simulink model "Bossi_Emanuele_EE460S3D_R99"  (R2025a)
settings: Solver=FixedStepDiscrete  StartTime=0.0  StopTime=120  FixedStep=dt0  RelTol=1e-3  EnableMultiTasking=on
PostLoadFcn:
  | %Set the size for the model
  | set_param(gcs,'Location',[10 10 1270 970])
  | %Set the zoom factor for the model
  | set_param(gcs,'ZoomFactor','100')
InitFcn:
  | tic
  | Bossi_Emanuele_EE460_Final
  | INIT_S3D_01
StartFcn:
  | tend0=toc;
  | tic;
StopFcn:
  | tend=toc;
  | disp(['Simulation time = ' num2str(tout(end)) ' sec'])
  | disp(['Real time = ' num2str(tend) ' sec'])
  | title('DONE')
  | SCORE=round((max(0,120-tout(end)-tend0))*4+10*(40-FuelBurned)+sum(100*double(PDONE)-100*double(PDONE<.5)));
  | PlotS3D(PlotInput);
  | text(15,22,['S: ' num2str(SCORE)]);
  | % Reset color scheme back to normal defaults
  | figure()
  | blkwhitebg('w');
  | close
values from neighbouring files (symbols this model uses):
  A_obs = [ 0  1  0  0  0  0 ... (first row only)    [Bossi_Emanuele_EE460_Final.m]
  B_obs = [ 0     0     0 ... (first row only)    [Bossi_Emanuele_EE460_Final.m]
  C_obs = [ 1 0 0 0 0 0 ... (first row only)    [Bossi_Emanuele_EE460_Final.m]
  d2r = pi/180    (= 0.0174532925199)    [INIT_S3D_01.m]
  D_obs = [ 0     0     0 ... (first row only)    [Bossi_Emanuele_EE460_Final.m]
  dt = 0.01    [INIT_S3D_01.m]
  dt0 = 0.001    [INIT_S3D_01.m]
  fr = 100    [INIT_S3D_01.m]
  G = [1,  1, -1, -1,  0,  0,  0,  0 ... (first row only)    [Bossi_Emanuele_EE460_Final.m]
  G_obs = eye(6)    [Bossi_Emanuele_EE460_Final.m]
  HM_S = 250    [INIT_S3D_01.m]
  HM_U = 500    [INIT_S3D_01.m]
  J = Jbase+JC0+JF+M*(Xcg^2+Ycg^2)    [INIT_S3D_01.m]
  Jbase = JC1+4*Ja+2*Ma*da^2+2*Ma*db^2    [INIT_S3D_01.m]
  JC0 = MC0/2    (= 10.2101761242)    [INIT_S3D_01.m]
  Kdtheta = 2 * zeta_th * wn_th * J_eff    [Bossi_Emanuele_EE460_Final.m]
  Kdtheta_fail = 2 * zeta_th_fail * wn_th_fail * J_eff    [Bossi_Emanuele_EE460_Final.m]
  Kdx = 2 * zeta_xy * wn_xy * M_eff    [Bossi_Emanuele_EE460_Final.m]
  Kdx_fail = 2 * zeta_xy_fail * wn_xy_fail * M_eff    [Bossi_Emanuele_EE460_Final.m]
  Kdy = 2 * zeta_xy * wn_xy * M_eff    [Bossi_Emanuele_EE460_Final.m]
  Kdy_fail = 2 * zeta_xy_fail * wn_xy_fail * M_eff    [Bossi_Emanuele_EE460_Final.m]
  Kptheta = J_eff * wn_th^2    [Bossi_Emanuele_EE460_Final.m]
  Kptheta_fail = J_eff * wn_th_fail^2    [Bossi_Emanuele_EE460_Final.m]
  Kpx = M_eff * wn_xy^2    [Bossi_Emanuele_EE460_Final.m]
  Kpx_fail = M_eff * wn_xy_fail^2    [Bossi_Emanuele_EE460_Final.m]
  Kpy = M_eff * wn_xy^2    [Bossi_Emanuele_EE460_Final.m]
  Kpy_fail = M_eff * wn_xy_fail^2    [Bossi_Emanuele_EE460_Final.m]
  L13 = sqrt(10)    [INIT_S3D_01.m]
  L24 = sqrt(6.25)    [INIT_S3D_01.m]
  LVL = LVL12    [INIT_S3D_01.m]
  M = MC+M1+M2+M3+M4+4*Ma    [INIT_S3D_01.m]
  M1 = LVL.M1    [INIT_S3D_01.m]
  M2 = LVL.M2    [INIT_S3D_01.m]
  M3 = LVL.M3    [INIT_S3D_01.m]
  M4 = LVL.M4    [INIT_S3D_01.m]
  max_qddot = [max_qddot_x; max_qddot_y; max_qddot_theta]    [Bossi_Emanuele_EE460_Final.m]
  mdti = (1/300)    (= 0.00333333333333)    [INIT_S3D_01.m]
  P = [1  1 -1 -1  0  0  0  0 ... (first row only)    [Bossi_Emanuele_EE460_Final.m]
  Pdata = [LVL.P1 LVL.P2 LVL.P3 LVL.P4]    [INIT_S3D_01.m]    (also in PlotS3D.m = R*[xt1;yt1+[0 3*tt*TV(idx-13)*TSIG(idx-13) 0]])
  PTvec = [Pdata(:,1);Pdata(:,2);Pdata(:,3);Pdata(:,4) ... (first row only)    [INIT_S3D_01.m]
  Q_obs = eye(6)    [Bossi_Emanuele_EE460_Final.m]
  r2d = 180/pi    (= 57.2957795131)    [INIT_S3D_01.m]
  r_bang = 0.5    [Bossi_Emanuele_EE460_Final.m]
  Sconfig = 1    [Bossi_Emanuele_EE460_Final.m]
  SLIM = [-100 100 ... (first row only)    [INIT_S3D_01.m]
  SQ = [.005 .01 .004 .005 .01 .004 .02 .01 .4]'    [INIT_S3D_01.m]
  SSF = 1./SQ    [INIT_S3D_01.m]
  tau = 0.5    [Bossi_Emanuele_EE460_Final.m]
  TOLdata = [LVL.P1tol LVL.P2tol LVL.P3tol LVL.P4tol]    [INIT_S3D_01.m]
  ULIM = [[Umin Umax];0 0;0 0]    [INIT_S3D_01.m]
undefined symbols (not defined in the file or in its folder): den_lp, den_lp2, DiscIntNeverNeededParam, dt1_bang_3, dt2_bang_3, dtc_bang_3, num_lp, num_lp2, q0_1
libraries: simulink x87, matrix_library x4, sl3dlib x1, aerolibutil x1, aerolibanimutils x1
(part 8 of 8)

== system Bossi_Emanuele_EE460S3D_R99/S3D_Plant/ThrusterValues/HealthMonitoring/DetectFailures/Subsystem9 ==
  UCMD : Inport
  U : Inport  Port=2
  Abs : Abs  SaturateOnIntegerOverflow=off
  Compare To Constant : simulink/Logic and Bit Operations/Compare To Constant  relop=>=  const=HM_U  OutDataTypeStr=boolean
  Constant : Constant  Value=0
  Constant1 : Constant
  Logical Operator : Logic  Operator=OR  AllPortsSameDT=off  OutDataTypeStr=boolean
  Signal Specification : SignalSpecification  Dimensions=[1]
  Signal Specification1 : SignalSpecification  Dimensions=[1]
  Sum : Sum  Inputs=|+-
  Sum1 : Sum  Inputs=++|
  Switch : Switch  Criteria=u2 > Threshold  Threshold=.4  SaturateOnIntegerOverflow=off  InputSameDT=off
  Unit Delay1 : UnitDelay  SampleTime=dt0  HasFrameUpgradeWarning=on
  Unit Delay2 : UnitDelay  SampleTime=dt0  HasFrameUpgradeWarning=on
  Out1 : Outport
  wires:
  Abs/1 -> Switch/2
  Signal Specification1/1 -> Sum/2
  Signal Specification/1 -> Sum/1
  Constant/1 -> Switch/3
  Sum1/1 -> Switch/1
  Unit Delay1/1 -> Sum1/1
  Constant1/1 -> Sum1/2
  U/1 -> Signal Specification1/1
  Logical Operator/1 -> Unit Delay2/1, Out1/1
  Compare To Constant/1 -> Logical Operator/1
  Switch/1 -> Unit Delay1/1, Compare To Constant/1
  UCMD/1 -> Signal Specification/1
  Unit Delay2/1 -> Logical Operator/2
  Sum/1 -> Abs/1

== system Bossi_Emanuele_EE460S3D_R99/ControlLaw/Command/AutoMode/BangBang_cmd/Precomputations/ComputeBCBTimes ==
  CurrentPosition1 : Inport
  In2 : Inport  Port=2
  FinalPosition1 : Inport  Port=3
  CurrentVelocity : Inport  Port=4
  Bus Creator : BusCreator  Inputs=3
  Bus Creator1 : BusCreator  Inputs=6
  Bus Selector : BusSelector  OutputSignals=FinalPosition,TriggeredPosition,a
  Constant : Constant  Value=r_bang  SampleTime=dt
  Constant1 : Constant
  Constant3 : Constant  Value=r_bang  SampleTime=dt
  DeltaQ : Subsystem
  Demux : Demux  Outputs=3
  Demux1 : Demux  Outputs=3
  Demux2 : Demux  Outputs=3
  Gain : Gain  Gain=2
  Max : MinMax  Function=max  Inputs=3
  Product : Product
  Product1 : Product
  RecomputeAccelerations : Subsystem
  Subsystem : Subsystem
  Sum1 : Sum  Inputs=|++
  Sum2 : Sum  Inputs=++|
  Sum3 : Sum  Inputs=++|
  Out4 : Outport
  Out1 : Outport  Port=2
  Out3 : Outport  Port=3
  Acc : Outport  Port=4
  wires:
  CurrentPosition1/1 -> Bus Creator/1
  In2/1 -> Bus Creator/2  "a"
  FinalPosition1/1 -> Bus Creator/3
  Bus Creator/1 -> Bus Selector/1
  Bus Selector/1 -> Demux1/1  "<FinalPosition>"
  Bus Selector/2 -> Demux2/1  "<TriggeredPosition>"
  DeltaQ/1(DeltaQ) -> RecomputeAccelerations/1(DeltaQ), Subsystem/2(DeltaQ)  "DeltaQ"
  Constant/1 -> Sum1/1
  Constant1/1 -> Sum1/2
  Bus Selector/3 -> Subsystem/3(Acc), Gain/1  "<a>"
  Sum1/1 -> Product/2
  Product/1 -> Subsystem/4(Den)  "rPlusOne"
  Subsystem/1(Out1) -> Demux/1
  Demux/2 -> Max/2
  Demux/1 -> Max/1
  Demux/3 -> Max/3
  Max/1 -> Product1/1, Sum2/2, RecomputeAccelerations/3(dt1), Sum3/1, Out1/1  "dt"
  Constant3/1 -> Product1/2
  Sum2/1 -> Out4/1  "TF"
  Product1/1 -> Sum3/2  "dtc"
  Sum3/1 -> Out3/1, Sum2/1  "DtPlusDtc"
  RecomputeAccelerations/1(Acc) -> Acc/1
  Demux1/1 -> Bus Creator1/1
  Demux1/2 -> Bus Creator1/2
  Demux1/3 -> Bus Creator1/3
  Demux2/1 -> Bus Creator1/4
  Demux2/2 -> Bus Creator1/5
  Demux2/3 -> Bus Creator1/6
  Bus Creator1/1 -> DeltaQ/1(In1)  "positions"
  Gain/1 -> Product/1
  CurrentVelocity/1 -> RecomputeAccelerations/2(v0), Subsystem/1(CurrentVelocity)

== system Bossi_Emanuele_EE460S3D_R99/ControlLaw/Command/AutoMode/BangBang_cmd/Precomputations/VariableTimer ==
  In1 : Inport
  Constant : Constant  Value=dt
  DetectTFchange : Subsystem
  Logical Operator : Logic  Operator=OR  AllPortsSameDT=off  OutDataTypeStr=boolean
  Relational Operator : RelationalOperator  Operator=<=  OutDataTypeStr=boolean  RndMeth=Simplest  InputSameDT=off
  Sum : Sum  Inputs=|++
  Switch : Switch  Criteria=u2 > Threshold  SaturateOnIntegerOverflow=off  InputSameDT=off
  Unit Delay1 : UnitDelay  SampleTime=dt  HasFrameUpgradeWarning=on
  Unit Delay2 : UnitDelay  InitialCondition=-dt  SampleTime=dt  HasFrameUpgradeWarning=on
  Time_sec : Outport
  wires:
  Unit Delay2/1 -> Sum/2
  Sum/1 -> Relational Operator/2, Switch/3
  Constant/1 -> Sum/1
  Logical Operator/1 -> Switch/2
  Switch/1 -> Time_sec/1, Unit Delay1/1, Unit Delay2/1  "Time_sec"
  DetectTFchange/1(Out1) -> Switch/1
  Unit Delay1/1 -> DetectTFchange/1(In1)  "TimeZ_sec"
  DetectTFchange/2(Out2) -> Logical Operator/1
  In1/1 -> DetectTFchange/2(In3), Relational Operator/1
  Relational Operator/1 -> Logical Operator/2  "Reset1"

== system Bossi_Emanuele_EE460S3D_R99/ControlLaw/Command/AutoMode/BangBang_cmd/ThetaTargetCorrector/AngleWrapper ==
  In1 : Inport
  Atan2 : Trigonometry  Operator=atan2
  Cos : Trigonometry  Operator=cos
  Gain : Gain  Gain=180/pi
  Gain6 : Gain  Gain=pi/180
  Sin : Trigonometry
  Out1 : Outport
  wires:
  Gain6/1 -> Cos/1, Sin/1
  In1/1 -> Gain6/1
  Atan2/1 -> Gain/1
  Gain/1 -> Out1/1  "WrappedAngle_deg"
  Sin/1 -> Atan2/1
  Cos/1 -> Atan2/2

== system Bossi_Emanuele_EE460S3D_R99/ControlLaw/Command/InitialPoint/BangBang_cmd/Precomputations/ComputeBCBTimes ==
  CurrentPosition1 : Inport
  In2 : Inport  Port=2
  Abs : Abs  SaturateOnIntegerOverflow=off
  Bus Creator : BusCreator  Inputs=3
  Bus Creator1 : BusCreator  Inputs=6
  Bus Selector : BusSelector  OutputSignals=FinalPosition,TriggeredPosition,a
  Constant : Constant  Value=r_bang  SampleTime=dt
  Constant1 : Constant
  Constant2 : Constant  Value=0.5  SampleTime=dt
  Constant3 : Constant  Value=r_bang  SampleTime=dt
  Constant4 : Constant  Value=[0; 0; 0]  SampleTime=dt
  DeltaQ : Subsystem
  Demux : Demux  Outputs=3
  Demux1 : Demux  Outputs=3
  Demux2 : Demux  Outputs=3
  Divide : Product  Inputs=*/
  Math Function : Math  Operator=pow
  Max : MinMax  Function=max  Inputs=3
  Product : Product
  Product1 : Product
  RecomputeAccelerations : Subsystem
  Sum1 : Sum  Inputs=|++
  Sum2 : Sum  Inputs=++|
  Sum3 : Sum  Inputs=++|
  Out4 : Outport
  Out1 : Outport  Port=2
  Out3 : Outport  Port=3
  Acc : Outport  Port=4
  wires:
  CurrentPosition1/1 -> Bus Creator/1
  In2/1 -> Bus Creator/2  "a"
  Bus Creator/1 -> Bus Selector/1
  Bus Selector/1 -> Demux1/1  "<FinalPosition>"
  Bus Selector/2 -> Demux2/1  "<TriggeredPosition>"
  DeltaQ/1(Out1) -> RecomputeAccelerations/1(In1), Divide/1  "DeltaQ"
  Constant/1 -> Sum1/1
  Constant1/1 -> Sum1/2
  Bus Selector/3 -> Product/1  "<a>"
  Sum1/1 -> Product/2
  Product/1 -> Divide/2  "rPlusOne"
  Constant2/1 -> Math Function/2
  Divide/1 -> Abs/1
  Math Function/1 -> Demux/1
  Demux/2 -> Max/2
  Demux/1 -> Max/1
  Demux/3 -> Max/3
  Max/1 -> Product1/1, Sum2/2, RecomputeAccelerations/2(In3), Sum3/1, Out1/1  "dt"
  Constant3/1 -> Product1/2
  Sum2/1 -> Out4/1  "TF"
  Product1/1 -> Sum3/2  "dtc"
  Sum3/1 -> Out3/1, Sum2/1  "DtPlusDtc"
  RecomputeAccelerations/1(Acc) -> Acc/1
  Demux1/1 -> Bus Creator1/1
  Demux1/2 -> Bus Creator1/2
  Demux1/3 -> Bus Creator1/3
  Demux2/1 -> Bus Creator1/4
  Demux2/2 -> Bus Creator1/5
  Demux2/3 -> Bus Creator1/6
  Bus Creator1/1 -> DeltaQ/1(In1)  "positions"
  Abs/1 -> Math Function/1
  Constant4/1 -> Bus Creator/3  "FinalPosition"

== system Bossi_Emanuele_EE460S3D_R99/ControlLaw/Command/InitialPoint/BangBang_cmd/Precomputations/VariableTimer ==
  In1 : Inport
  Constant : Constant  Value=dt
  DetectTFchange : Subsystem
  Logical Operator : Logic  Operator=OR  AllPortsSameDT=off  OutDataTypeStr=boolean
  Relational Operator : RelationalOperator  Operator=<=  OutDataTypeStr=boolean  RndMeth=Simplest  InputSameDT=off
  Sum : Sum  Inputs=|++
  Switch : Switch  Criteria=u2 > Threshold  SaturateOnIntegerOverflow=off  InputSameDT=off
  Unit Delay1 : UnitDelay  SampleTime=dt  HasFrameUpgradeWarning=on
  Unit Delay2 : UnitDelay  InitialCondition=-dt  SampleTime=dt  HasFrameUpgradeWarning=on
  Time_sec : Outport
  wires:
  Unit Delay2/1 -> Sum/2
  Sum/1 -> Relational Operator/2, Switch/3
  Constant/1 -> Sum/1
  Logical Operator/1 -> Switch/2
  Switch/1 -> Time_sec/1, Unit Delay1/1, Unit Delay2/1  "Time_sec"
  DetectTFchange/1(Out1) -> Switch/1
  Unit Delay1/1 -> DetectTFchange/1(In1)  "TimeZ_sec"
  DetectTFchange/2(Out2) -> Logical Operator/1
  In1/1 -> DetectTFchange/2(In3), Relational Operator/1
  Relational Operator/1 -> Logical Operator/2  "Reset1"

== system Bossi_Emanuele_EE460S3D_R99/ControlLaw/Command/InitialPoint/BangBang_cmd/ThetaTargetCorrector/AngleWrapper ==
  In1 : Inport
  Atan2 : Trigonometry  Operator=atan2
  Cos : Trigonometry  Operator=cos
  Gain : Gain  Gain=180/pi
  Gain6 : Gain  Gain=pi/180
  Sin : Trigonometry
  Out1 : Outport
  wires:
  Gain6/1 -> Cos/1, Sin/1
  In1/1 -> Gain6/1
  Atan2/1 -> Gain/1
  Gain/1 -> Out1/1  "WrappedAngle_deg"
  Sin/1 -> Atan2/1
  Cos/1 -> Atan2/2

== system Bossi_Emanuele_EE460S3D_R99/ControlLaw/Command/AutoMode/BangBang_cmd/Precomputations/ComputeBCBTimes/DeltaQ ==
  In1 : Inport
  Bus Selector1 : BusSelector  OutputSignals=signal1,signal4,signal2,signal5,signal3,signal6
  Display : Display
  Sum : Sum  Inputs=|+-
  Sum4 : Sum  Inputs=|+-
  ThetaTargetCorrector : Subsystem
  Vector Concatenate : Concatenate  NumInputs=3
  DeltaQ : Outport
  wires:
  Bus Selector1/4 -> Sum4/2  "<signal5>"
  Bus Selector1/3 -> Sum4/1  "<signal2>"
  Sum4/1 -> Vector Concatenate/2  "DeltaY"
  Bus Selector1/1 -> Sum/1  "<signal1>"
  Bus Selector1/2 -> Sum/2  "<signal4>"
  Bus Selector1/5 -> ThetaTargetCorrector/1(In2)  "<signal3>"
  ThetaTargetCorrector/1(Out1) -> Vector Concatenate/3  "qc"
  Bus Selector1/6 -> ThetaTargetCorrector/2(In1)  "<signal6>"
  Sum/1 -> Display/1, Vector Concatenate/1  "DeltaX"
  In1/1 -> Bus Selector1/1
  Vector Concatenate/1 -> DeltaQ/1  "DeltaQ"

== system Bossi_Emanuele_EE460S3D_R99/ControlLaw/Command/AutoMode/BangBang_cmd/Precomputations/ComputeBCBTimes/RecomputeAccelerations ==
  DeltaQ : Inport
  v0 : Inport  Port=2
  dt1 : Inport  Port=3
  Constant : Constant  Value=r_bang  SampleTime=dt
  Constant1 : Constant  Value=r_bang  SampleTime=dt
  Constant2 : Constant  Value=2
  Constant3 : Constant
  Constant4 : Constant  Value=2
  Divide : Product  Inputs=*/
  Pow : Math  Operator=pow  SignedPower=on  RndMeth=Zero
  Product : Product  Inputs=3
  Product1 : Product
  Sum : Sum  Inputs=|++
  Sum1 : Sum  Inputs=|+-
  Sum2 : Sum  Inputs=|++
  Acc : Outport
  wires:
  Divide/1 -> Acc/1  "a"
  Constant2/1 -> Sum/1
  Constant/1 -> Sum/2
  Sum/1 -> Product/2
  v0/1 -> Product/1
  dt1/1 -> Pow/1, Product/3
  DeltaQ/1 -> Sum1/1
  Sum1/1 -> Divide/1
  Product/1 -> Sum1/2
  Constant1/1 -> Sum2/2
  Constant3/1 -> Sum2/1
  Sum2/1 -> Product1/2
  Pow/1 -> Product1/1
  Constant4/1 -> Pow/2
  Product1/1 -> Divide/2

== system Bossi_Emanuele_EE460S3D_R99/ControlLaw/Command/AutoMode/BangBang_cmd/Precomputations/ComputeBCBTimes/Subsystem ==
  CurrentVelocity : Inport
  DeltaQ : Inport  Port=2
  Acc : Inport  Port=3
  Den : Inport  Port=4
  Abs : Abs  SaturateOnIntegerOverflow=off
  Bus Creator : BusCreator  Inputs=2
  Bus Selector : BusSelector  OutputSignals=NegVelZero,TwoPlusR,NegVelZero,TwoPlusR
  Constant : Constant  Value=r_bang  SampleTime=dt
  Constant1 : Constant  Value=2
  Constant2 : Constant  Value=2
  Constant3 : Constant  Value=2
  Constant4 : Constant  Value=r_bang  SampleTime=dt
  Constant5 : Constant
  Constant6 : Constant  Value=0.5
  Divide : Product  Inputs=*/
  Exp : Math  Operator=pow
  Exp1 : Math  Operator=pow
  Gain : Gain  Gain=-1
  Gain1 : Gain  Gain=4
  Pow : Math  Operator=pow  SignedPower=on  RndMeth=Zero
  Product : Product
  Product1 : Product
  Product2 : Product  Inputs=3
  Sum : Sum  Inputs=|++
  Sum1 : Sum  Inputs=|++
  Sum2 : Sum  Inputs=|++|
  Sum3 : Sum  Inputs=|++
  Out1 : Outport
  wires:
  CurrentVelocity/1 -> Gain/1
  Constant/1 -> Sum/1
  Constant1/1 -> Sum/2
  Gain/1 -> Bus Creator/1  "NegVelZero"
  Sum/1 -> Bus Creator/2  "TwoPlusR"
  Bus Creator/1 -> Bus Selector/1
  Bus Selector/1 -> Product/1  "<NegVelZero>"
  Bus Selector/2 -> Product/2  "<TwoPlusR>"
  Bus Selector/3 -> Exp/1  "<NegVelZero>"
  Constant2/1 -> Exp/2
  Bus Selector/4 -> Exp1/1  "<TwoPlusR>"
  Constant3/1 -> Exp1/2
  Exp/1 -> Product1/1
  Exp1/1 -> Product1/2
  Product1/1 -> Sum1/1
  Constant5/1 -> Sum2/2
  Constant4/1 -> Sum2/1
  Acc/1 -> Gain1/1
  Gain1/1 -> Product2/1
  Sum2/1 -> Product2/2  "TwoPlusR"
  DeltaQ/1 -> Product2/3
  Product2/1 -> Sum1/2
  Sum1/1 -> Abs/1
  Abs/1 -> Pow/1
  Constant6/1 -> Pow/2
  Pow/1 -> Sum3/2
  Product/1 -> Sum3/1
  Sum3/1 -> Divide/1
  Den/1 -> Divide/2
  Divide/1 -> Out1/1  "t1"

== system Bossi_Emanuele_EE460S3D_R99/ControlLaw/Command/AutoMode/BangBang_cmd/Precomputations/VariableTimer/DetectTFchange ==
  In1 : Inport
  In3 : Inport  Port=2
  Constant : Constant  Value=0
  Relational Operator1 : RelationalOperator  Operator=~=  OutDataTypeStr=boolean  RndMeth=Simplest  InputSameDT=off
  Switch3 : Switch  Criteria=u2 > Threshold  SaturateOnIntegerOverflow=off  InputSameDT=off
  Unit Delay : UnitDelay  InitialCondition=-dt  SampleTime=dt  HasFrameUpgradeWarning=on
  Out1 : Outport
  Out2 : Outport  Port=2
  wires:
  Switch3/1 -> Out1/1  "ResetValue"
  In3/1 -> Relational Operator1/1, Unit Delay/1
  Unit Delay/1 -> Relational Operator1/2
  Relational Operator1/1 -> Out2/1, Switch3/2  "Reset2"
  In1/1 -> Switch3/3
  Constant/1 -> Switch3/1

== system Bossi_Emanuele_EE460S3D_R99/ControlLaw/Command/InitialPoint/BangBang_cmd/Precomputations/ComputeBCBTimes/DeltaQ ==
  In1 : Inport
  Bus Selector1 : BusSelector  OutputSignals=signal1,signal4,signal2,signal5,signal3,signal6
  Display : Display
  Sum : Sum  Inputs=|+-
  Sum4 : Sum  Inputs=|+-
  ThetaTargetCorrector : Subsystem
  Vector Concatenate : Concatenate  NumInputs=3
  Out1 : Outport
  wires:
  Bus Selector1/4 -> Sum4/2  "<signal5>"
  Bus Selector1/3 -> Sum4/1  "<signal2>"
  Sum4/1 -> Vector Concatenate/2  "DeltaY"
  Bus Selector1/1 -> Sum/1  "<signal1>"
  Bus Selector1/2 -> Sum/2  "<signal4>"
  Bus Selector1/5 -> ThetaTargetCorrector/1(In2)  "<signal3>"
  ThetaTargetCorrector/1(Out1) -> Vector Concatenate/3  "qc"
  Bus Selector1/6 -> ThetaTargetCorrector/2(In1)  "<signal6>"
  Sum/1 -> Display/1, Vector Concatenate/1  "DeltaX"
  In1/1 -> Bus Selector1/1
  Vector Concatenate/1 -> Out1/1  "DeltaQ"

== system Bossi_Emanuele_EE460S3D_R99/ControlLaw/Command/InitialPoint/BangBang_cmd/Precomputations/ComputeBCBTimes/RecomputeAccelerations ==
  In1 : Inport
  In3 : Inport  Port=2
  Constant : Constant  Value=r_bang  SampleTime=dt
  Constant1 : Constant
  Constant2 : Constant  Value=2
  Constant3 : Constant  Value=0.000000001
  Divide : Product  Inputs=*/
  Pow : Math  Operator=pow  SignedPower=on  RndMeth=Zero
  Product : Product
  Sum1 : Sum  Inputs=|++
  Switch : Switch  Criteria=u2 ~= 0  SaturateOnIntegerOverflow=off  InputSameDT=off
  Acc : Outport
  wires:
  Sum1/1 -> Product/2
  Constant1/1 -> Sum1/2
  Constant/1 -> Sum1/1
  In3/1 -> Pow/1
  Product/1 -> Switch/1, Switch/2  "rPlusOne"
  In1/1 -> Divide/1
  Pow/1 -> Product/1
  Constant2/1 -> Pow/2
  Divide/1 -> Acc/1  "a"
  Switch/1 -> Divide/2
  Constant3/1 -> Switch/3

== system Bossi_Emanuele_EE460S3D_R99/ControlLaw/Command/InitialPoint/BangBang_cmd/Precomputations/VariableTimer/DetectTFchange ==
  In1 : Inport
  In3 : Inport  Port=2
  Constant : Constant  Value=0
  Relational Operator1 : RelationalOperator  Operator=~=  OutDataTypeStr=boolean  RndMeth=Simplest  InputSameDT=off
  Switch3 : Switch  Criteria=u2 > Threshold  SaturateOnIntegerOverflow=off  InputSameDT=off
  Unit Delay : UnitDelay  InitialCondition=-dt  SampleTime=dt  HasFrameUpgradeWarning=on
  Out1 : Outport
  Out2 : Outport  Port=2
  wires:
  Switch3/1 -> Out1/1  "ResetValue"
  In3/1 -> Relational Operator1/1, Unit Delay/1
  Unit Delay/1 -> Relational Operator1/2
  Relational Operator1/1 -> Out2/1, Switch3/2  "Reset2"
  In1/1 -> Switch3/3
  Constant/1 -> Switch3/1

== system Bossi_Emanuele_EE460S3D_R99/ControlLaw/Command/AutoMode/BangBang_cmd/Precomputations/ComputeBCBTimes/DeltaQ/ThetaTargetCorrector ==
  In2 : Inport
  In1 : Inport  Port=2
  AngleWrapper : Subsystem
  Sum : Sum  Inputs=|+-
  Out1 : Outport
  wires:
  In2/1 -> Sum/1
  In1/1 -> Sum/2
  Sum/1 -> AngleWrapper/1(In1)  "theta_deg"
  AngleWrapper/1(Out1) -> Out1/1

== system Bossi_Emanuele_EE460S3D_R99/ControlLaw/Command/InitialPoint/BangBang_cmd/Precomputations/ComputeBCBTimes/DeltaQ/ThetaTargetCorrector ==
  In2 : Inport
  In1 : Inport  Port=2
  AngleWrapper : Subsystem
  Sum : Sum  Inputs=|+-
  Out1 : Outport
  wires:
  In2/1 -> Sum/1
  In1/1 -> Sum/2
  Sum/1 -> AngleWrapper/1(In1)  "theta_deg"
  AngleWrapper/1(Out1) -> Out1/1

== system Bossi_Emanuele_EE460S3D_R99/ControlLaw/Command/AutoMode/BangBang_cmd/Precomputations/ComputeBCBTimes/DeltaQ/ThetaTargetCorrector/AngleWrapper ==
  In1 : Inport
  Atan2 : Trigonometry  Operator=atan2
  Cos : Trigonometry  Operator=cos
  Gain : Gain  Gain=180/pi
  Gain6 : Gain  Gain=pi/180
  Sin : Trigonometry
  Out1 : Outport
  wires:
  Gain6/1 -> Cos/1, Sin/1
  In1/1 -> Gain6/1
  Atan2/1 -> Gain/1
  Gain/1 -> Out1/1  "WrappedAngle_deg"
  Sin/1 -> Atan2/1
  Cos/1 -> Atan2/2

== system Bossi_Emanuele_EE460S3D_R99/ControlLaw/Command/InitialPoint/BangBang_cmd/Precomputations/ComputeBCBTimes/DeltaQ/ThetaTargetCorrector/AngleWrapper ==
  In1 : Inport
  Atan2 : Trigonometry  Operator=atan2
  Cos : Trigonometry  Operator=cos
  Gain : Gain  Gain=180/pi
  Gain6 : Gain  Gain=pi/180
  Sin : Trigonometry
  Out1 : Outport
  wires:
  Gain6/1 -> Cos/1, Sin/1
  In1/1 -> Gain6/1
  Atan2/1 -> Gain/1
  Gain/1 -> Out1/1  "WrappedAngle_deg"
  Sin/1 -> Atan2/1
  Cos/1 -> Atan2/2
